simulink model "PLLGGGGG"  (R2025a)
settings: Solver=VariableStepAuto  StartTime=0.0  StopTime=10  RelTol=1e-3
libraries: commdigbbndpm3 x2, commchan3 x1, commrflib2 x1, commrandsrc3 x1
settings Model: Creator=ulma5  LastModifiedBy=LaL
settings RTWCC: GPUComputeCapability=3.5

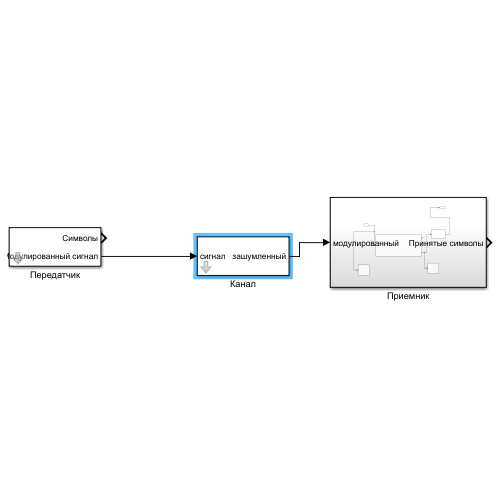
[thumbnail: Simulink's stored preview of the top-level diagram]
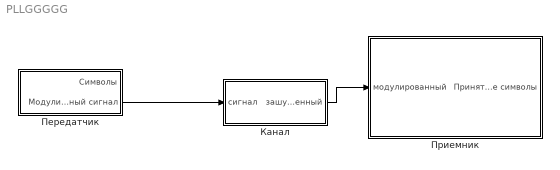
== system PLLGGGGG ==
  Канал : Subsystem  mask{T_symb=25000, param_sdvig=0.0001, phase_offset=30}
      mask prompts: T_symb "Символьная скорость"; param_sdvig "Параметр сдвига"; phase_offset "Сдвиг фазы (deg)"
  Передатчик : Subsystem  mask{T_symb=25000}
      mask prompts: T_symb "симв скорость"
  Приемник : Subsystem
  wires:
  Передатчик/2(Модулированный сигнал) -> Канал/1(сигнал)
  Канал/1(зашумленный) -> Приемник/1(модулированный)

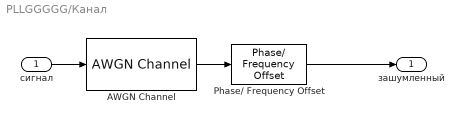
== system PLLGGGGG/Канал ==
  сигнал : Inport
  AWGN Channel : commchan3/AWGN Channel  LegacyMode=off  NoiseMethod="Signal to noise ratio  (SNR)"  noiseMode="Signal to noise ratio  (SNR)"  EbNo=10  EsNo=10  SNR=40  BitsPerSymbol=1  SignalPower=1  SpecifySymbolPeriod=off  SamplesPerSymbol=1  SymbolPeriod=1  VarianceSource=Parameter  Variance=1  RandomStream=Global stream  Seed=67  SimulateUsing=Interpreted execution
  Phase/ Frequency Offset : commrflib2/Phase// Frequency Offset  phaseOffset=phase_offset  freqPort=off  freqOffset=T_symb*param_sdvig
  зашумленный : Outport
  wires:
  сигнал/1 -> AWGN Channel/1
  AWGN Channel/1 -> Phase/ Frequency Offset/1
  Phase/ Frequency Offset/1 -> зашумленный/1

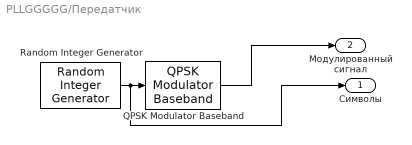
== system PLLGGGGG/Передатчик ==
  QPSK Modulator Baseband : commdigbbndpm3/QPSK Modulator Baseband  InType=Integer  Enc=Gray  Ph=pi/4  outDtype=double  outWordLen=16  outUDDataType=sfix(16)  outFracLenMode=Best precision  outFracLen=15  outDataTypeStr=double  outLastDataTypeStr=double
      settings: LibrarySourceBlock=|
      | commhdldigbbndpm/QPSK
      | Modulator
      | Baseband
  Random Integer Generator : commrandsrc3/Random Integer Generator  SetSize=4  SeedSource=Auto  Seed=0  SampleTime=1/T_symb  SamplesPerFrame=1  OutputDataType=double  SimulateUsing=Interpreted execution
  Символы : Outport
  Модулированный сигнал : Outport  Port=2
  wires:
  Random Integer Generator/1 -> Символы/1, QPSK Modulator Baseband/1
  QPSK Modulator Baseband/1 -> Модулированный сигнал/1

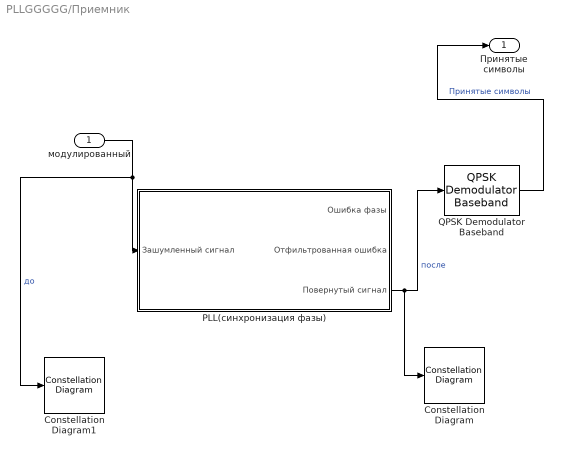
== system PLLGGGGG/Приемник ==
  модулированный : Inport
  Constellation Diagram : ConstellationDiagram  WindowPosition=[382.000000,84.000000,600.000000,600.000000,]  ScopeFrameLocation=window  DefaultConfigurationName=comm.scopes.ConstellationDiagramBlockCfg
  Constellation Diagram1 : ConstellationDiagram  WindowPosition=[243.000000,155.000000,600.000000,600.000000,]  ScopeFrameLocation=window  SymbolsToDisplaySource=Property  SymbolsToDisplay=100  XLimits=[-1.46,1.46]  YLimits=[-1.38,1.38]  AxesLimits=[-1.38,1.38]  DefaultConfigurationName=comm.scopes.ConstellationDiagramBlockCfg
  PLL(синхронизация фазы) : Subsystem
  QPSK Demodulator Baseband : commdigbbndpm3/QPSK Demodulator Baseband  OutType=Integer  DecType=Hard decision  VarSource=Dialog  Variance=1  Dec=Gray  Ph=pi/4  outDtype1=Inherit via internal rule  outDtype2=Inherit via internal rule  derotateFactorWordLen=16  derotateFactorDataTypeStr=Inherit: Same word length as input  derotateFactorLastDataTypeStr=Inherit: Same word length as input
      settings: LibrarySourceBlock=|
      | commhdldigbbndpm/QPSK
      | Demodulator
      | Baseband
  Принятые символы : Outport
  wires:
  QPSK Demodulator Baseband/1 -> Принятые символы/1  "Принятые символы"
  PLL(синхронизация фазы)/3(Повернутый сигнал) -> Constellation Diagram/1, QPSK Demodulator Baseband/1  "после"
  модулированный/1 -> Constellation Diagram1/1, PLL(синхронизация фазы)/1(Зашумленный сигнал)  "до"

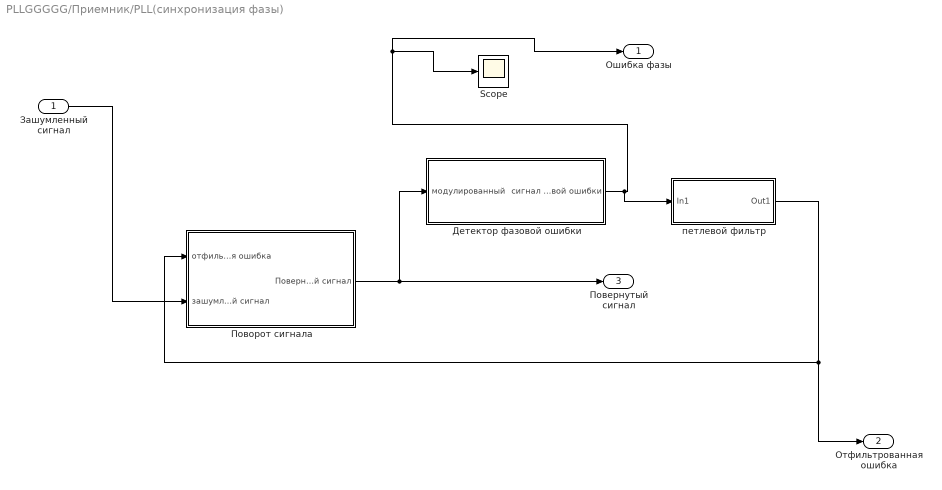
== system PLLGGGGG/Приемник/PLL(синхронизация фазы) ==
  Зашумленный сигнал : Inport
  Scope : Scope
      settings: ActiveDisplayYMinimum=0.48589  ActiveDisplayYMaximum=0.56246
  Детектор фазовой ошибки : Subsystem
  Поворот сигнала : Subsystem
  петлевой фильтр : Subsystem  mask{BW=0.0001, dzeta=1/sqrt(2), N=1, Kd=1}
      mask prompts: BW "нормалированная ширина полосы"; dzeta "дэмпинг фактор фильтра"; N "количество отсчетов на символ"; Kd "коэффициент детектора"
  Ошибка фазы : Outport
  Отфильтрованная ошибка : Outport  Port=2
  Повернутый сигнал : Outport  Port=3
  wires:
  Детектор фазовой ошибки/1(сигнал фазовой ошибки) -> петлевой фильтр/1(In1), Ошибка фазы/1, Scope/1
  Зашумленный сигнал/1 -> Поворот сигнала/2(зашумленный сигнал)
  Поворот сигнала/1(Повернутый сигнал) -> Детектор фазовой ошибки/1(модулированный), Повернутый сигнал/1
  петлевой фильтр/1(Out1) -> Поворот сигнала/1(отфильтрованная ошибка), Отфильтрованная ошибка/1

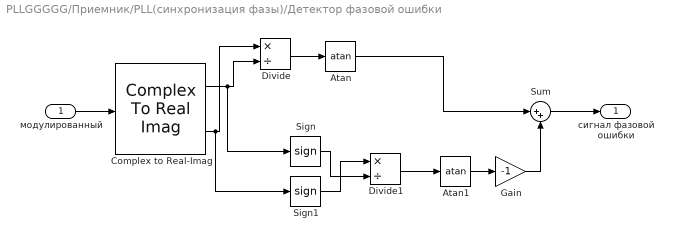
== system PLLGGGGG/Приемник/PLL(синхронизация фазы)/Детектор фазовой ошибки ==
  модулированный : Inport
  Atan : Trigonometry  Operator=atan
  Atan1 : Trigonometry  Operator=atan
  Complex to Real-Imag : ComplexToRealImag
  Divide : Product  Inputs=*/
  Divide1 : Product  Inputs=*/
  Gain : Gain  Gain=-1
  Sign : Signum
  Sign1 : Signum
  Sum : Sum  Inputs=|++
  сигнал фазовой ошибки : Outport
  wires:
  модулированный/1 -> Complex to Real-Imag/1
  Complex to Real-Imag/1 -> Sign/1, Divide/2
  Complex to Real-Imag/2 -> Sign1/1, Divide/1
  Divide/1 -> Atan/1
  Sign1/1 -> Divide1/1
  Sign/1 -> Divide1/2
  Divide1/1 -> Atan1/1
  Atan1/1 -> Gain/1
  Atan/1 -> Sum/1
  Gain/1 -> Sum/2
  Sum/1 -> сигнал фазовой ошибки/1

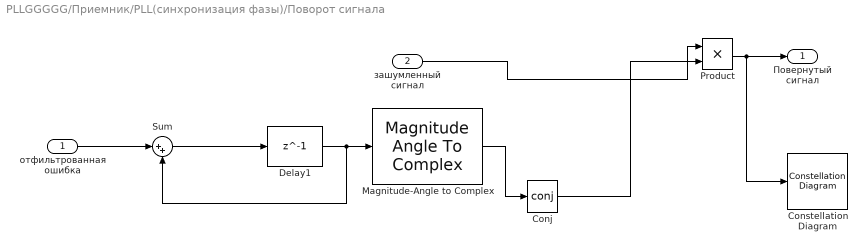
== system PLLGGGGG/Приемник/PLL(синхронизация фазы)/Поворот сигнала ==
  отфильтрованная ошибка : Inport
  зашумленный сигнал : Inport  Port=2
  Conj : Math  Operator=conj
  Constellation Diagram : ConstellationDiagram  WindowPosition=[614.000000,167.000000,600.000000,600.000000,]  ScopeFrameLocation=window  SymbolsToDisplaySource=Property  SymbolsToDisplay=100  XLimits=[-2.86,1.89]  YLimits=[-2.66,1.82]  AxesLimits=[-2.66,1.82]  DefaultConfigurationName=comm.scopes.ConstellationDiagramBlockCfg
  Delay1 : Delay  DelayLength=1  InitialCondition=0  UseCircularBuffer=on
  Magnitude-Angle to Complex : MagnitudeAngleToComplex  Input=Angle  ConstantPart=1
  Product : Product
  Sum : Sum  Inputs=|++
  Повернутый сигнал : Outport
  wires:
  Sum/1 -> Delay1/1
  Delay1/1 -> Sum/2, Magnitude-Angle to Complex/1
  отфильтрованная ошибка/1 -> Sum/1
  зашумленный сигнал/1 -> Product/1
  Product/1 -> Повернутый сигнал/1, Constellation Diagram/1
  Magnitude-Angle to Complex/1 -> Conj/1
  Conj/1 -> Product/2

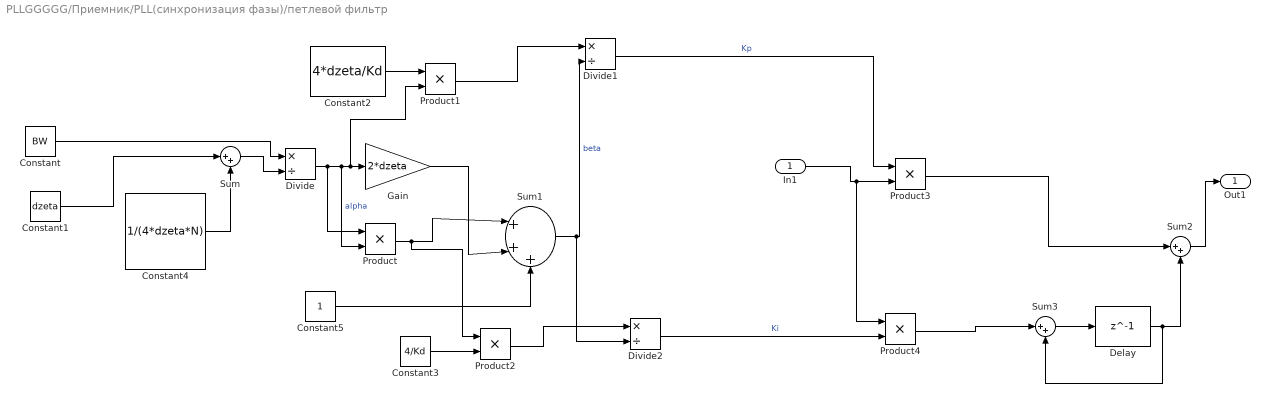
== system PLLGGGGG/Приемник/PLL(синхронизация фазы)/петлевой фильтр ==
  In1 : Inport
  Constant : Constant  Value=BW
  Constant1 : Constant  Value=dzeta
  Constant2 : Constant  Value=4*dzeta/Kd
  Constant3 : Constant  Value=4/Kd
  Constant4 : Constant  Value=1/(4*dzeta*N)
  Constant5 : Constant
  Delay : Delay  DelayLength=1  InitialCondition=0  UseCircularBuffer=on
  Divide : Product  Inputs=*/
  Divide1 : Product  Inputs=*/
  Divide2 : Product  Inputs=*/
  Gain : Gain  Gain=2*dzeta
  Product{,1..4} (5 alike) : Product
  Sum : Sum  Inputs=|++
  Sum1 : Sum  Inputs=|+++
  Sum2 : Sum  Inputs=|++
  Sum3 : Sum  Inputs=|++
  Out1 : Outport
  wires:
  Constant1/1 -> Sum/1
  Constant4/1 -> Sum/2
  Sum/1 -> Divide/2
  Constant/1 -> Divide/1
  Divide/1 -> Product/1, Product/2, Product1/2, Gain/1  "alpha"
  Constant5/1 -> Sum1/3
  Gain/1 -> Sum1/2
  Product/1 -> Product2/1, Sum1/1
  Sum1/1 -> Divide2/2, Divide1/2  "beta"
  Constant2/1 -> Product1/1
  Product1/1 -> Divide1/1
  Divide1/1 -> Product3/1  "Kp"
  Constant3/1 -> Product2/2
  Product2/1 -> Divide2/1
  Divide2/1 -> Product4/2  "Ki"
  In1/1 -> Product4/1, Product3/2
  Sum2/1 -> Out1/1
  Product4/1 -> Sum3/1
  Sum3/1 -> Delay/1
  Delay/1 -> Sum2/2, Sum3/2
  Product3/1 -> Sum2/1
